simulink model "aerodynamic_model_V1_2_Wrench"  (R2025b)
settings: Solver=ode4  StartTime=0.0  StopTime=0.3  FixedStep=Ts  RelTol=1e-3
InitFcn:
  | % Run initial_main.m first to load Ad,As,Tq_prop,Tq_mass,...
values from neighbouring files (symbols this model uses):
  alpha_du0_v_tail_L = trim_aero_ic.v_tail_L.alpha_du0    [initial_main_V1_1.m]
  alpha_du0_v_tail_R = trim_aero_ic.v_tail_R.alpha_du0    [initial_main_V1_1.m]
  alpha_du0_wing_L = trim_aero_ic.wing_L.alpha_du0    [initial_main_V1_1.m]
  alpha_du0_wing_R = trim_aero_ic.wing_R.alpha_du0    [initial_main_V1_1.m]
  As = sys_sd.A    [initial_main_V1_1.m]
  BladePitch_deg = 34    [initial_main_V1_1.m]
  Bs = sys_sd.B    [initial_main_V1_1.m]
  Cs = sys_sd.C    [initial_main_V1_1.m]
  ctrl_delta_lim_deg = strips.delta_lim_deg    [initial_main_V1_1.m]
  ctrl_map_aileron_L = aero.wing_L.map_aileron(:)    [initial_main_V1_1.m]
  ctrl_map_aileron_R = aero.wing_R.map_aileron(:)    [initial_main_V1_1.m]
  ctrl_map_tail_L = aero.v_tail_L.map_tail(:)    [initial_main_V1_1.m]
  ctrl_map_tail_R = aero.v_tail_R.map_tail(:)    [initial_main_V1_1.m]
  Ds = sys_sd.D    [initial_main_V1_1.m]
  I_cg_b = R_sb * I_cg_m * R_sb.'    [aeroelastic.m]    (also in initial_main_V1_1.m = grav.I_cg_b)
  I_cg_b_inv = R_sb * I_cg_m_inv * R_sb.'    [aeroelastic.m]    (also in initial_main_V1_1.m = grav.I_cg_b_inv)
  m_node = zeros(n_id, 1)    [aeroelastic.m]    (also in generate_pullup_load_cloud.m = evalin('base', 'm_node(:)'); initial_main_V1_1.m = nodal.m_node)
  m_total_kg = evalin('base', 'm_total_kg')    [generate_pullup_load_cloud.m]    (also in initial_main_V1_1.m = grav.m_total_kg)
  n_modes = size(Phi, 2)    [aeroelastic.m]    (also in initial_main_V1_1.m = n_rigid + n_elastic)
  ones_1_tail = ones(1, size(r_cg2ac_b_v_tail_L, 2))    [initial_main_V1_1.m]
  ones_1_wing = ones(1, size(r_cg2ac_b_wing_L, 2))    [initial_main_V1_1.m]
  Phi = evalin('base', 'Phi')    [generate_pullup_load_cloud.m]    (also in initial_main_V1_1.m = strips.Phi)
  polar_alpha_deg = polar.alpha_deg(:).'    [initial_main_V1_1.m]
  polar_CD = polar.CD(:).'    [initial_main_V1_1.m]
  polar_CDp = polar.CDp(:).'    [initial_main_V1_1.m]
  polar_CL = polar.CL(:).'    [initial_main_V1_1.m]
  polar_CM = polar.CM(:).'    [initial_main_V1_1.m]
  r_cg2ac_b_v_tail_L = R_sb * aero.v_tail_L.r_ac_s    [initial_main_V1_1.m]
  r_cg2ac_b_v_tail_R = R_sb * aero.v_tail_R.r_ac_s    [initial_main_V1_1.m]
  r_cg2ac_b_wing_L = R_sb * aero.wing_L.r_ac_s    [initial_main_V1_1.m]
  r_cg2ac_b_wing_R = R_sb * aero.wing_R.r_ac_s    [initial_main_V1_1.m]
  r_cg2kink_b = eng.r_cg2kink_b    [initial_main_V1_1.m]
  r_cg2node_b = aeroelastic.node_arms(nodes, 'R_sb', R_sb).r_cg2node_b    [initial_main_V1_1.m]
  surface_nodes = aeroelastic.surface_load_nodes(nodes)    [initial_main_V1_1.m]
  T_aero2W = aeroelastic.wing_aileron_to_W(strips).T    [initial_main_V1_1.m]
  T_prop2W = load_maps.T_prop2W    [initial_main_V1_1.m]
  Tq_mass = load_maps.Tq_mass    [initial_main_V1_1.m]
  trim_Attitude_rad0 = trim_default.Attitude_rad0    [initial_main_V1_1.m]
  trim_Omega_b0 = trim_default.Omega_b0    [initial_main_V1_1.m]
  trim_Position0 = trim_default.Position0    [initial_main_V1_1.m]
  trim_Velocity_b0 = trim_default.Velocity_b0    [initial_main_V1_1.m]
  Ts = 0.001    [initial_main_V1_1.m]
  U = 55    [initial_main_V1_1.m]
  v_tail_cant_rad = deg2rad(v_tail_cant_deg)    [initial_main_V1_1.m]
  W_mass_g = grav.W_mass    [initial_main_V1_1.m]
  x0_structure = trim_default.x0_structure    [initial_main_V1_1.m]
  x0_wagner_v_tail_L = trim_aero_ic.v_tail_L.x0_wagner    [initial_main_V1_1.m]
  x0_wagner_v_tail_R = trim_aero_ic.v_tail_R.x0_wagner    [initial_main_V1_1.m]
  x0_wagner_wing_L = trim_aero_ic.wing_L.x0_wagner    [initial_main_V1_1.m]
  x0_wagner_wing_R = trim_aero_ic.wing_R.x0_wagner    [initial_main_V1_1.m]
undefined symbols (not defined in the file or in its folder): Ad_v_tail_L, Ad_v_tail_R, Ad_wing_L, Ad_wing_R, Bd_v_tail_L, Bd_v_tail_R, Bd_wing_L, Bd_wing_R, c_over_2U_v_tail_L, c_over_2U_v_tail_R, c_over_2U_wing_L, c_over_2U_wing_R, Cd_v_tail_L, Cd_v_tail_R, Cd_wing_L, Cd_wing_R, Dd_v_tail_L, Dd_v_tail_R, Dd_wing_L, Dd_wing_R, G_du_v_tail_L, G_du_v_tail_R, G_du_wing_L, G_du_wing_R, polar_aileron_alpha_deg, polar_aileron_dCD, polar_aileron_dCL, polar_aileron_dCM, polar_aileron_delta_deg, polar_ruddervator_alpha_deg, polar_ruddervator_dCD, polar_ruddervator_dCL, polar_ruddervator_dCM, polar_ruddervator_delta_deg, qS_strip_v_tail_L, qS_strip_v_tail_R, qS_strip_wing_L, qS_strip_wing_R, qSc_strip_v_tail_L, qSc_strip_v_tail_R, qSc_strip_wing_L, qSc_strip_wing_R, T_m2b_v_tail_L, T_m2b_v_tail_R, T_m2b_wing_L, T_m2b_wing_R, T_m2h_v_tail_L, T_m2h_v_tail_R, T_m2h_wing_L, T_m2h_wing_R, Tq_CM_v_tail_L, Tq_CM_v_tail_R, Tq_CM_wing_L, Tq_CM_wing_R, Tq_D_v_tail_L, Tq_D_v_tail_R, Tq_D_wing_L, Tq_D_wing_R, Tq_v_tail_L, Tq_v_tail_R ... (+2)
libraries: Prop_gryo x12, matrix_library x2
(part 1 of 6)
settings Model: Creator=someone  LastModifiedBy=someone
settings DataIOCC: ExternalInput=trim_input_dataset  LoadExternalInput=on

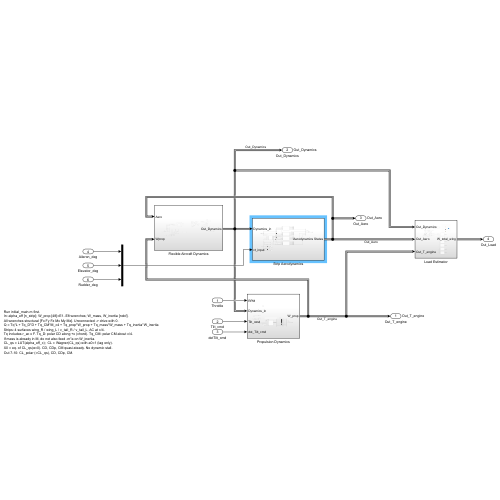
[thumbnail: Simulink's stored preview of the top-level diagram]
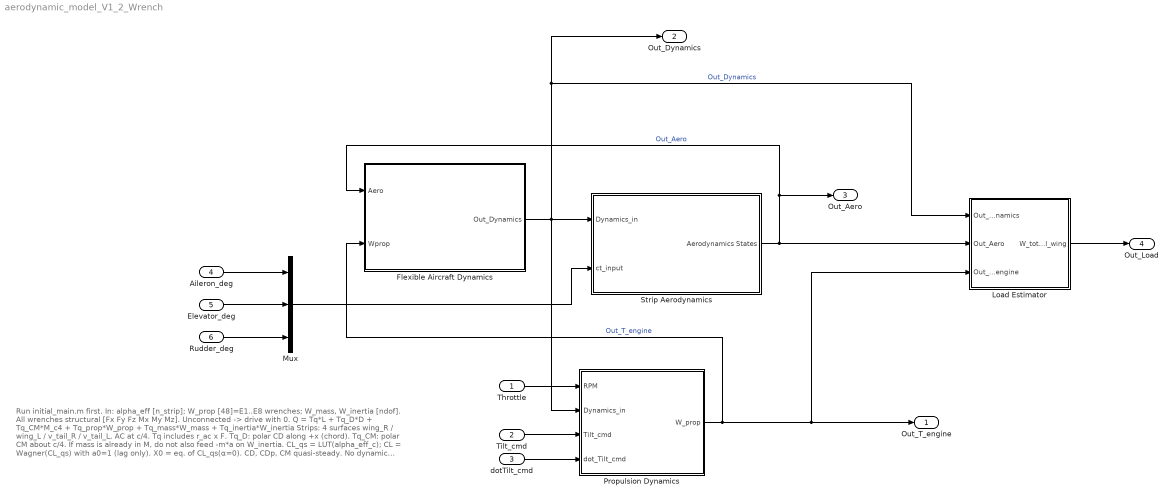
== system aerodynamic_model_V1_2_Wrench ==
  note: Run initial_main.m first.
      | In: alpha_eff [n_strip]; W_prop [48]=E1..E8 wrenches; W_mass, W_inertia [ndof].
      | All wrenches structural [Fx Fy Fz Mx My Mz]. Unconnected -> drive with 0.
      | Q = Tq*L + Tq_D*D + Tq_CM*M_c4 + Tq_prop*W_prop + Tq_mass*W_mass + Tq_inertia*W_inertia
      | Strips: 4 surfaces wing_R / wing_L / v_tail_R / v_tail_L, AC at c/4.
      | Tq includes r_ac x F. Tq_D: polar CD along +x (chord). Tq_CM: polar CM about c/4.
      | If mass is already in M, do not also feed -m*a on W_inertia.
      | CL_qs = LUT(alpha_eff_c);  CL = Wagner(CL_qs) with a0=1 (lag only).
      | X0 = eq. of CL_qs(α=0). CD, CDp, CM quasi-steady. No dynamic stall.
      | Out 7-10: CL_polar (=CL_qs), CD, CDp, CM.
  Throttle : Inport  PortDimensions=8
  Tilt_cmd : Inport  Port=2  PortDimensions=8
  dotTilt_cmd : Inport  Port=3  PortDimensions=8
  Aileron_deg : Inport  Port=4
  Elevator_deg : Inport  Port=5
  Rudder_deg : Inport  Port=6
  Flexible Aircraft Dynamics : Subsystem
  Load Estimator : Subsystem
  Mux : Mux  Inputs=3
  Propulsion Dynamics : Subsystem
  Strip Aerodynamics : Subsystem
  Out_T_engine : Outport  SignalName=Out_T_engine
  Out_Dynamics : Outport  Port=2  SignalName=Out_Dynamics
  Out_Aero : Outport  Port=3  SignalName=Out_Aero
  Out_Load : Outport  Port=4
  wires:
  Throttle/1 -> Propulsion Dynamics/1(RPM)
  Tilt_cmd/1 -> Propulsion Dynamics/3(Tilt_cmd)
  dotTilt_cmd/1 -> Propulsion Dynamics/4(dot_Tilt_cmd)
  Flexible Aircraft Dynamics/1(Out_Dynamics) -> Out_Dynamics/1, Load Estimator/1(Out_Dynamics), Strip Aerodynamics/1(Dynamics_in), Propulsion Dynamics/2(Dynamics_in)  "Out_Dynamics"
  Strip Aerodynamics/1(Aerodynamics States) -> Out_Aero/1, Flexible Aircraft Dynamics/1(Aero), Load Estimator/2(Out_Aero)  "Out_Aero"
  Propulsion Dynamics/1(W_prop) -> Load Estimator/3(Out_T_engine), Out_T_engine/1, Flexible Aircraft Dynamics/2(Wprop)  "Out_T_engine"
  Aileron_deg/1 -> Mux/1
  Rudder_deg/1 -> Mux/3
  Mux/1 -> Strip Aerodynamics/2(ct_input)
  Elevator_deg/1 -> Mux/2
  Load Estimator/1(W_total_wing) -> Out_Load/1

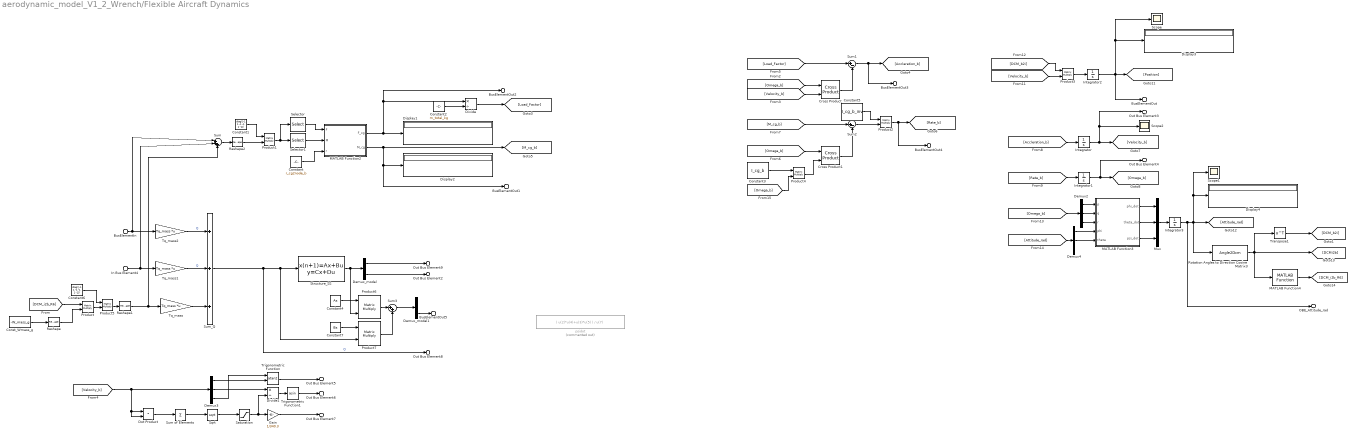
== system aerodynamic_model_V1_2_Wrench/Flexible Aircraft Dynamics ==
  BusElementIn : Inport  PortName=Aero  Element=W_aero_S
  In Bus Element4 : Inport  Port=2  PortName=Wprop  Element=W_m
  Const_Wmass_g : Constant  Value=-W_mass_g
  Constant : Constant  Value=r_cg2node_b
  Constant1 : Constant  Value=diag([-1 1 -1 -1 1 -1])
  Constant2 : Constant  Value=m_total_kg
  Constant3 : Constant  Value=I_cg_b
  Constant4 : Constant  Value=As
  Constant5 : Constant  Value=I_cg_b_inv
  Constant6 : Constant  Value=diag([-1 1 -1 -1 1 -1])
  Constant7 : Constant  Value=Bs
  Cross Product : matrix_library/Cross Product
  Cross Product1 : matrix_library/Cross Product
  Demux2 : Demux  Outputs=3
  Demux3 : Demux  Outputs=3
  Demux4 : Demux  Outputs=3
  Demux_modal : Demux  Outputs=[n_modes n_modes]
  Demux_modal1 : Demux  Outputs=[n_modes n_modes]
  Display{1..4} (4 alike) : Display
  Divide : Product  Inputs=*/
  Divide1 : Product  Inputs=*/
  Dot Product : DotProduct  OutDataTypeStr=Inherit: Inherit via internal rule
  Gain : Gain  Gain=1/340.3
  Integrator : Integrator  InitialCondition=trim_Velocity_b0
  Integrator1 : Integrator  InitialCondition=trim_Omega_b0
  Integrator2 : Integrator  InitialCondition=trim_Position0
  Integrator3 : Integrator  InitialCondition=trim_Attitude_rad0
  MATLAB Function2 : MATLAB Function  TreatAsAtomicUnit=on
  MATLAB Function3 : MATLAB Function  TreatAsAtomicUnit=on
  MATLAB Function4 : Prop_gryo/Prop1/MATLAB Function  SystemSampleTime=-1  VariantActivationTime=update diagram  EmptyChoice=off  PassThrough=off  PassThroughVariantControl=(default)  EmptyChoiceVariantControl=(default)  AllowFlexibleInterface=on  Latency=0  AutoFrameSizeCalculation=off
  Mux : Mux  Inputs=3
  Product{,1..7} (8 alike) : Product  Multiplication=Matrix(*)
  Reshape : Reshape  OutputDimensionality=Customize  OutputDimensions=[6 89]
  Reshape1 : Reshape
  Reshape2 : Reshape  OutputDimensionality=Customize  OutputDimensions=[6 89]
  Rotation Angles to Direction Cosine Matrix3 : Angle2Dcm
      settings: AttributesFormatString=Rotation Order: %<rotationOrder>
  Saturation : Saturate  UpperLimit=inf  LowerLimit=1e-6
  Scope : Scope
      settings: ActiveDisplayYMinimum=-1  ActiveDisplayYMaximum=1
  Scope1 : Scope
      settings: ActiveDisplayYMinimum=-0.70675522606206342  ActiveDisplayYMaximum=0.36695629334776858
  Scope2 : Scope
      settings: ActiveDisplayYMinimum=-1  ActiveDisplayYMaximum=1  DataLoggingVariableName=ScopeData2
  Selector : Selector  NumberOfDimensions=2  InputPortWidth=3  IndexOptions=Index vector (dialog),Index vector (dialog)  Indices=[1:3],[1:89]  OutputSizes=1,1
  Selector1 : Selector  NumberOfDimensions=2  InputPortWidth=3  IndexOptions=Index vector (dialog),Index vector (dialog)  Indices=[4:6],[1:89]  OutputSizes=1,1
  Sqrt : Sqrt
  Structure_SS : DiscreteStateSpace  A=As  B=Bs  C=Cs  D=Ds  InitialCondition=x0_structure  SampleTime=Ts
  Sum : Sum  Inputs=|+++
  Sum of Elements : Sum  Inputs=+
  Sum1 : Sum  Inputs=|+-
  Sum2 : Sum  Inputs=|+-
  Sum3 : Sum  Inputs=|++
  Sum_Q : Sum  Inputs=+++
  Tq_mass : Gain  Gain=Tq_mass  Multiplication=Matrix(K*u)
  Tq_mass1 : Gain  Gain=Tq_mass  Multiplication=Matrix(K*u)
  Tq_mass2 : Gain  Gain=Tq_mass  Multiplication=Matrix(K*u)
  Transpose1 : Math  Operator=transpose
  Trigonometric Function : Trigonometry  Operator=atan2
  Trigonometric Function1 : Trigonometry  Operator=asin
  psidot : Fcn  Commented=on  Expr=( u(2)*u(4)+u(3)*u(5) ) / u(7)
  Out Bus Element2 : Outport  PortName=Out_Dynamics  Element=elastic_m_velocity
  Out Bus Element3 : Outport  PortName=Out_Dynamics  Element=Velocity_b
  Out Bus Element4 : Outport  PortName=Out_Dynamics  Element=Omega_b
  Out Bus Element5 : Outport  PortName=Out_Dynamics  Element=Alpha
  Out Bus Element6 : Outport  PortName=Out_Dynamics  Element=Beta
  Out Bus Element7 : Outport  PortName=Out_Dynamics  Element=mach
  Out Bus Element8 : Outport  PortName=Out_Dynamics  Element=Q
  Out Bus Element9 : Outport  PortName=Out_Dynamics  Element=elastic_displacement
  OBE_Attitude_rad : Outport  PortName=Out_Dynamics  Element=Attitude_rad
  BusElementOut : Outport  PortName=Out_Dynamics  Element=Position
  BusElementOut1 : Outport  PortName=Out_Dynamics  Element=M_cg
  BusElementOut2 : Outport  PortName=Out_Dynamics  Element=F_cg
  BusElementOut3 : Outport  PortName=Out_Dynamics  Element=Acc_b
  BusElementOut4 : Outport  PortName=Out_Dynamics  Element=Rate_b
  BusElementOut5 : Outport  PortName=Out_Dynamics  Element=elastic_acc
  wires:
  Dot Product/1 -> Sum of Elements/1
  [Velocity_b] -> Demux3/1, Dot Product/2, Dot Product/1
  Demux3/3 -> Trigonometric Function/1
  Sum_Q/1 -> Product7/2, Structure_SS/1, Out Bus Element8/1  "Q"
  In Bus Element4/1 -> Tq_mass1/1, Sum/2
  Demux_modal/2 -> Out Bus Element2/1
  Demux_modal/1 -> Out Bus Element9/1
  Tq_mass/1 -> Sum_Q/3
  Sum of Elements/1 -> Sqrt/1
  Demux3/2 -> Divide1/1
  Structure_SS/1 -> Product6/2, Demux_modal/1
  Divide1/1 -> Trigonometric Function1/1
  Demux3/1 -> Trigonometric Function/2
  Const_Wmass_g/1 -> Reshape/1
  Sqrt/1 -> Saturation/1
  Saturation/1 -> Gain/1, Divide1/2
  Trigonometric Function/1 -> Out Bus Element5/1
  Trigonometric Function1/1 -> Out Bus Element6/1
  Gain/1 -> Out Bus Element7/1
  Tq_mass1/1 -> Sum_Q/2  "Q"
  BusElementIn/1 -> Sum/1, Tq_mass2/1
  Tq_mass2/1 -> Sum_Q/1  "Q"
  [DCM_i2b_R6] -> Product/1
  Reshape/1 -> Product/2
  Product5/1 -> Reshape1/1
  Reshape1/1 -> Tq_mass/1, Sum/3
  Sum/1 -> Reshape2/1
  Reshape2/1 -> Product1/2
  Selector/1 -> MATLAB Function2/1(F)
  Selector1/1 -> MATLAB Function2/2(M)
  Constant/1 -> MATLAB Function2/3(r)
  Constant1/1 -> Product1/1
  Product1/1 -> Selector1/1, Selector/1
  MATLAB Function2/1(F_cg) -> BusElementOut2/1, Divide/1, Display1/1
  MATLAB Function2/2(M_cg) -> Display2/1, BusElementOut1/1, [M_cg_b]
  [Omega_b] -> Cross Product/1
  [Velocity_b] -> Cross Product/2
  [Load_Factor] -> Sum1/1
  Cross Product/1 -> Sum1/2
  Constant2/1 -> Divide/2
  Divide/1 -> [Load_Factor]
  Sum1/1 -> BusElementOut3/1, [Accleration_b]
  [Omega_b] -> Cross Product1/1
  Constant3/1 -> Product4/1
  [M_cg_b] -> Sum2/1
  Cross Product1/1 -> Sum2/2
  [Accleration_b] -> Integrator/1
  [Rate_b] -> Integrator1/1
  Integrator/1 -> Scope2/1, Out Bus Element3/1, [Velocity_b]
  Integrator1/1 -> Out Bus Element4/1, [Omega_b]
  Sum2/1 -> Product2/2
  Constant5/1 -> Product2/1
  Product2/1 -> BusElementOut4/1, [Rate_b]
  [Velocity_b] -> Product3/2
  [DCM_b2i] -> Product3/1
  Product3/1 -> Integrator2/1
  Integrator2/1 -> BusElementOut/1, Display3/1, Scope/1, [Position]
  Integrator3/1 -> Rotation Angles to Direction Cosine Matrix3/1, Scope1/1, Display4/1, [Attitude_rad], OBE_Attitude_rad/1
  [Omega_b] -> Demux2/1
  Demux2/1 -> MATLAB Function3/1(p)
  Demux2/2 -> MATLAB Function3/2(q)
  Demux2/3 -> MATLAB Function3/3(r)
  [Attitude_rad] -> Demux4/1
  Demux4/1 -> MATLAB Function3/4(phi)
  Demux4/2 -> MATLAB Function3/5(theta)
  Mux/1 -> Integrator3/1
  MATLAB Function3/1(phi_dot) -> Mux/1
  MATLAB Function3/2(theta_dot) -> Mux/2
  MATLAB Function3/3(psi_dot) -> Mux/3
  [Omega_b] -> Product4/2
  Product4/1 -> Cross Product1/2
  Rotation Angles to Direction Cosine Matrix3/1 -> Transpose1/1, MATLAB Function4/1, [DCMi2b]
  MATLAB Function4/1 -> [DCM_i2b_R6]
  Transpose1/1 -> [DCM_b2i]
  Constant6/1 -> Product5/1
  Product/1 -> Product5/2
  Product6/1 -> Sum3/1
  Product7/1 -> Sum3/2
  Constant4/1 -> Product6/1
  Constant7/1 -> Product7/1
  Sum3/1 -> Demux_modal1/1
  Demux_modal1/2 -> BusElementOut5/1

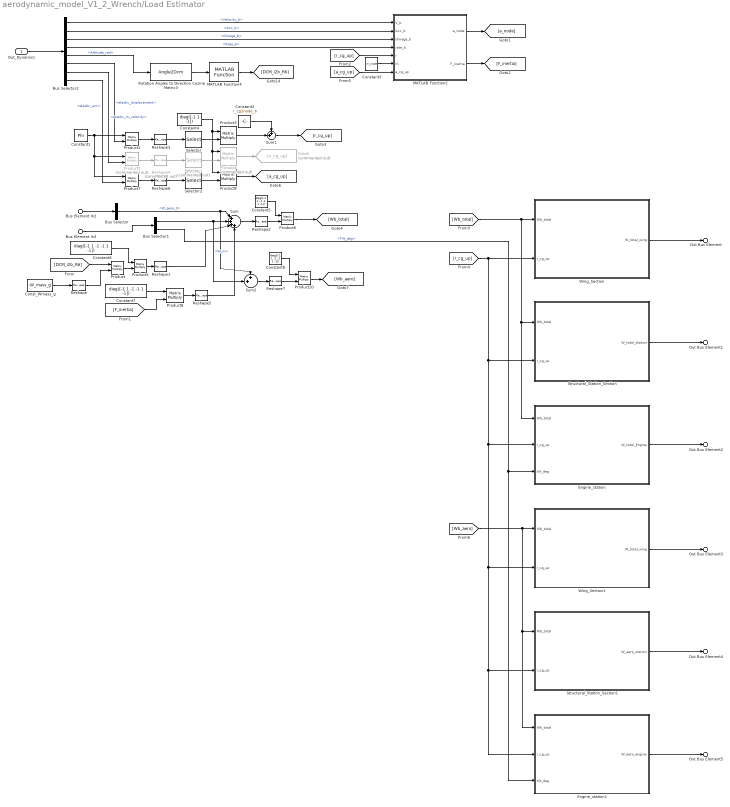
== system aerodynamic_model_V1_2_Wrench/Load Estimator ==
  Out_Dynamics : Inport
  Bus Element In2 : Inport  Port=2  PortName=Out_Aero
  Bus Element In3 : Inport  Port=3  PortName=Out_T_engine
  Bus Selector : BusSelector  OutputSignals=W_aero_S
  Bus Selector1 : BusSelector  OutputSignals=W_m,Tilt_deg
  Bus Selector2 : BusSelector  OutputSignals=Velocity_b,Acc_b,Omega_b,Rate_b,Attitude_rad,elastic_displacement,elastic_m_velocity,elastic_acc
  Const_Wmass_g : Constant  Value=-W_mass_g
  Constant1 : Constant  Value=Phi
  Constant2 : Constant  Value=r_cg2node_b
  Constant3 : Constant  Value=m_node
  Constant4 : Constant  Value=diag([-1 1 -1])
  Constant{5..8} (4 alike) : Constant  Value=diag([-1 1 -1 -1 1 -1])
  Engine_station : Subsystem
  Engine_station1 : Subsystem
  Goto5 : Goto  Commented=on  GotoTag=v_cg_up
  MATLAB Function2 : MATLAB Function  TreatAsAtomicUnit=on
  MATLAB Function4 : Prop_gryo/Prop1/MATLAB Function  SystemSampleTime=-1  VariantActivationTime=update diagram  EmptyChoice=off  PassThrough=off  PassThroughVariantControl=(default)  EmptyChoiceVariantControl=(default)  AllowFlexibleInterface=on  Latency=0  AutoFrameSizeCalculation=off
  Product{,1,3,5..10} (9 alike) : Product  Multiplication=Matrix(*)
  Product2 : Product  Commented=on  Multiplication=Matrix(*)
  Product4 : Product  Commented=on  Multiplication=Matrix(*)
  Reshape{,2..3,6..7} (5 alike) : Reshape  OutputDimensionality=Customize  OutputDimensions=[6 89]
  Reshape1 : Reshape
  Reshape4 : Reshape  Commented=on  OutputDimensionality=Customize  OutputDimensions=[6 89]
  Reshape5 : Reshape
  Rotation Angles to Direction Cosine Matrix3 : Angle2Dcm
      settings: AttributesFormatString=Rotation Order: %<rotationOrder>
  Selector : Selector  NumberOfDimensions=2  InputPortWidth=89  IndexOptions=Index vector (dialog),Index vector (dialog)  Indices=[1:3],[1:89]  OutputSizes=1,1
  Selector1 : Selector  Commented=on  NumberOfDimensions=2  InputPortWidth=89  IndexOptions=Index vector (dialog),Index vector (dialog)  Indices=[1:3],[1:89]  OutputSizes=1,1
  Selector2 : Selector  NumberOfDimensions=2  InputPortWidth=89  IndexOptions=Index vector (dialog),Index vector (dialog)  Indices=[1:3],[1:89]  OutputSizes=1,1
  Structural_Station_Section : Subsystem
  Structural_Station_Section1 : Subsystem
  Sum : Sum  Inputs=|++++
  Sum1 : Sum  Inputs=++|
  Sum2 : Sum  Inputs=++|
  Wing_Section : Subsystem
  Wing_Section1 : Subsystem
  Out Bus Element : Outport  PortName=W_total_wing  Element=W_total_wing
  Out Bus Element1 : Outport  PortName=W_total_wing  Element=W_total_station
  Out Bus Element2 : Outport  PortName=W_total_wing  Element=W_total_engine
  Out Bus Element3 : Outport  PortName=W_total_wing  Element=W_aero_wing
  Out Bus Element4 : Outport  PortName=W_total_wing  Element=W_aero_station
  Out Bus Element5 : Outport  PortName=W_total_wing  Element=W_aero_engine
  wires:
  Sum/1 -> Reshape2/1
  Bus Selector1/1 -> Sum2/2, Sum/2  "<W_m>"
  Bus Selector/1 -> Sum/1, Sum2/1  "<W_aero_S>"
  Reshape1/1 -> Sum/3
  Bus Element In2/1 -> Bus Selector/1
  Bus Element In3/1 -> Bus Selector1/1
  Reshape/1 -> Product/2
  Const_Wmass_g/1 -> Reshape/1
  [DCM_i2b_R6] -> Product/1
  Constant6/1 -> Product5/1
  Product5/1 -> Reshape1/1
  Product/1 -> Product5/2
  Out_Dynamics/1 -> Bus Selector2/1
  Bus Selector2/1 -> MATLAB Function2/1(V_b)  "<Velocity_b>"
  Bus Selector2/3 -> MATLAB Function2/3(Omega_b)  "<Omega_b>"
  Bus Selector2/2 -> MATLAB Function2/2(Acc_b)  "<Acc_b>"
  [r_cg_up] -> MATLAB Function2/5(r)
  Bus Selector2/4 -> MATLAB Function2/4(rate_b)  "<Rate_b>"
  Constant3/1 -> MATLAB Function2/6(m)
  Rotation Angles to Direction Cosine Matrix3/1 -> MATLAB Function4/1
  Bus Selector2/5 -> Rotation Angles to Direction Cosine Matrix3/1  "<Attitude_rad>"
  MATLAB Function4/1 -> [DCM_i2b_R6]
  MATLAB Function2/1(a_node) -> [a_node]
  MATLAB Function2/2(F_inertia) -> [F_inertia]
  Reshape5/1 -> Sum/4
  Bus Selector2/6 -> Product1/2  "<elastic_displacement>"
  Constant1/1 -> Product1/1, Product2/1, Product7/1
  Bus Selector2/7 -> Product2/2  "<elastic_m_velocity>"
  Product1/1 -> Reshape3/1
  Product2/1 -> Reshape4/1
  Reshape3/1 -> Selector/1
  Reshape4/1 -> Selector1/1
  Selector/1 -> Product3/2
  Constant4/1 -> Product8/1, Product4/1, Product3/1
  Selector1/1 -> Product4/2
  Constant2/1 -> Sum1/1
  Sum1/1 -> [r_cg_up]
  Product3/1 -> Sum1/2
  Product9/1 -> Reshape5/1
  Reshape2/1 -> Product6/2
  Product4/1 -> Goto5/1
  [a_cg_up] -> MATLAB Function2/7(a_cg_up)
  [Wb_total] -> Engine_station/1(Wb_total), Structural_Station_Section/1(Wb_total), Wing_Section/1(Wb_total)
  [r_cg_up] -> Structural_Station_Section/2(r_cg_up), Wing_Section1/2(r_cg_up), Engine_station1/2(r_cg_up), Structural_Station_Section1/2(r_cg_up), Engine_station/2(r_cg_up), Wing_Section/2(r_cg_up)
  Wing_Section/1(W_total_wing) -> Out Bus Element/1
  Structural_Station_Section/1(W_total_station) -> Out Bus Element1/1
  Engine_station/1(W_total_Engine) -> Out Bus Element2/1
  Bus Selector1/2 -> Engine_station/3(tilt_deg), Engine_station1/3(tilt_deg)  "<Tilt_deg>"
  Constant5/1 -> Product6/1
  Product6/1 -> [Wb_total]
  Product8/1 -> [a_cg_up]
  Selector2/1 -> Product8/2
  Reshape6/1 -> Selector2/1
  Product7/1 -> Reshape6/1
  Bus Selector2/8 -> Product7/2  "<elastic_acc>"
  [F_inertia] -> Product9/2
  Constant7/1 -> Product9/1
  Product10/1 -> [Wb_aero]
  Constant8/1 -> Product10/1
  Reshape7/1 -> Product10/2
  Sum2/1 -> Reshape7/1
  [Wb_aero] -> Wing_Section1/1(Wb_total), Engine_station1/1(Wb_total), Structural_Station_Section1/1(Wb_total)
  Wing_Section1/1(W_total_wing) -> Out Bus Element3/1
  Structural_Station_Section1/1(W_aero_station) -> Out Bus Element4/1
  Engine_station1/1(W_aero_engine) -> Out Bus Element5/1

== system aerodynamic_model_V1_2_Wrench/Propulsion Dynamics ==
  note: 根据体轴速度、加速度、引擎和铰链位置以及铰链轴和倾转角速率计算各个引擎体轴下绝对速度
  RPM : Inport  PortDimensions=8
  Dynamics_in : Inport  Port=2
  Tilt_cmd : Inport  Port=3  PortDimensions=8
  dot_Tilt_cmd : Inport  Port=4  PortDimensions=8
  BladePitch_deg : Constant  Value=BladePitch_deg
  Bus Selector : BusSelector  OutputSignals=signal1.Wb,signal2.Wb,signal3.Wb,signal4.Wb,signal5.Wb,signal6.Wb,signal7.Wb,signal8.Wb
  BusSel_Dynamic : BusSelector  OutputSignals=mach,Velocity_b,Omega_b
  Constant : Constant  Value=diag([-1 1 1 -1 1 1])
  Constant1 : Constant  Value=T_prop2W
  Constant4 : Constant  Commented=on  Value=(pi/2)*ones(8,1)
  Delay_Dynamic : UnitDelay  Commented=through  SampleTime=Ts  HasFrameUpgradeWarning=on
  Gain : Gain  Gain=1/60
  Mux1 : Mux  Inputs=8
  Product{,1..8} (9 alike) : Product  Multiplication=Matrix(*)
  Subsystem8 : Subsystem
  Out Bus Element1 : Outport  PortName=W_prop  Element=W_m
  BusElementOut : Outport  PortName=W_prop  Element=Tilt_deg
  wires:
  Dynamics_in/1 -> Delay_Dynamic/1
  Delay_Dynamic/1 -> BusSel_Dynamic/1
  BusSel_Dynamic/2 -> Subsystem8/3(Vb)  "<Velocity_b>"
  BusSel_Dynamic/3 -> Subsystem8/4(Omegab)  "<Omega_b>"
  RPM/1 -> [RPM], Gain/1
  Gain/1 -> [RPS]
  BladePitch_deg/1 -> [BladePitchAngle_DEG]
  Tilt_cmd/1 -> BusElementOut/1, Subsystem8/1(In1)
  dot_Tilt_cmd/1 -> Subsystem8/2(In2)
  [BladePitchAngle_DEG] -> Subsystem8/5(BladePitchAngle_DEG)
  [RPS] -> Subsystem8/6(RPS)
  Subsystem8/1(Prop) -> Bus Selector/1
  Constant/1 -> Product7/1, Product6/1, Product5/1, Product4/1, Product3/1, Product2/1, Product1/1, Product/1
  Bus Selector/8 -> Product7/2  "<Wb>"
  Bus Selector/7 -> Product6/2  "<Wb>"
  Bus Selector/6 -> Product5/2  "<Wb>"
  Bus Selector/5 -> Product4/2  "<Wb>"
  Bus Selector/4 -> Product3/2  "<Wb>"
  Bus Selector/3 -> Product2/2  "<Wb>"
  Bus Selector/2 -> Product1/2  "<Wb>"
  Product/1 -> Mux1/1
  Product1/1 -> Mux1/2
  Product2/1 -> Mux1/3
  Product3/1 -> Mux1/4
  Product4/1 -> Mux1/5
  Product5/1 -> Mux1/6
  Product6/1 -> Mux1/7
  Product7/1 -> Mux1/8
  Mux1/1 -> Product8/2
  Constant1/1 -> Product8/1
  Product8/1 -> Out Bus Element1/1
  Bus Selector/1 -> Product/2  "<Wb>"

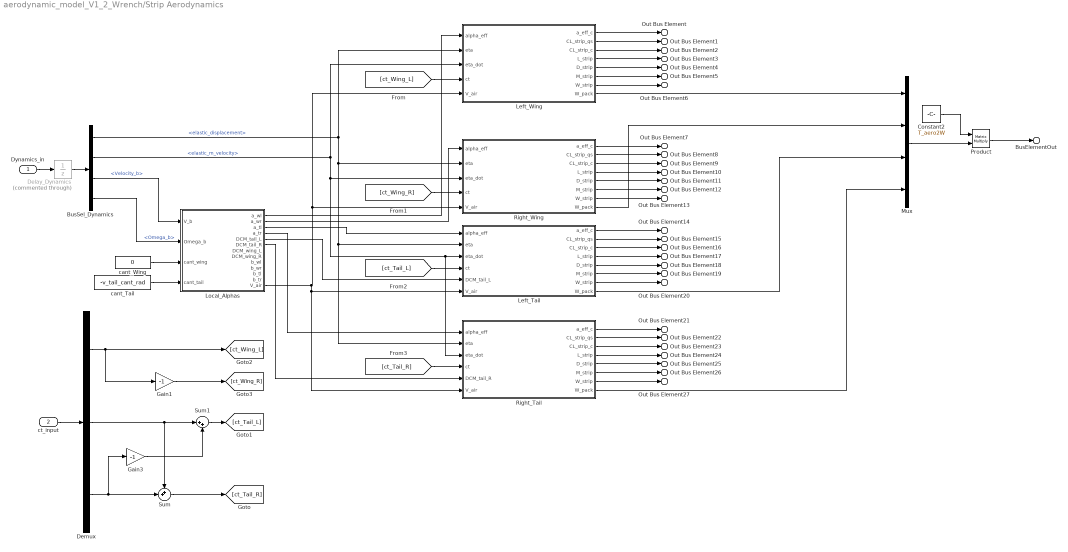
== system aerodynamic_model_V1_2_Wrench/Strip Aerodynamics ==
  Dynamics_in : Inport
  ct_input : Inport  Port=2
  BusSel_Dynamics : BusSelector  OutputSignals=elastic_displacement,elastic_m_velocity,Velocity_b,Omega_b
  Constant2 : Constant  Value=T_aero2W
  Delay_Dynamics : UnitDelay  Commented=through  SampleTime=Ts  HasFrameUpgradeWarning=on
  Demux : Demux  Outputs=3
  Gain1 : Gain  Gain=-1
  Gain3 : Gain  Gain=-1
  Left_Tail : Subsystem
  Left_Wing : Subsystem
  Local_Alphas : Subsystem
  Mux : Mux
  Product : Product  Multiplication=Matrix(*)
  Right_Tail : Subsystem
  Right_Wing : Subsystem
  Sum : Sum  Inputs=++|
  Sum1 : Sum  Inputs=|++
  cant_Tail : Constant  Value=-v_tail_cant_rad
  cant_Wing : Constant  Value=0
  Out Bus Element : Outport  PortName=Aerodynamics States  Element=a_eff_c_LW
  Out Bus Element1 : Outport  PortName=Aerodynamics States  Element=CL_strip_qs_LW
  Out Bus Element2 : Outport  PortName=Aerodynamics States  Element=CL_strip_c_LW
  Out Bus Element3 : Outport  PortName=Aerodynamics States  Element=L_strip_LW
  Out Bus Element4 : Outport  PortName=Aerodynamics States  Element=D_strip_LW
  Out Bus Element5 : Outport  PortName=Aerodynamics States  Element=M_strip_LW
  Out Bus Element6 : Outport  PortName=Aerodynamics States  Element=W_strip_LW
  Out Bus Element7 : Outport  PortName=Aerodynamics States  Element=a_eff_c_RW
  Out Bus Element8 : Outport  PortName=Aerodynamics States  Element=CL_strip_qs_RW
  Out Bus Element9 : Outport  PortName=Aerodynamics States  Element=CL_strip_c_RW
  Out Bus Element10 : Outport  PortName=Aerodynamics States  Element=L_strip_RW
  Out Bus Element11 : Outport  PortName=Aerodynamics States  Element=D_strip_RW
  Out Bus Element12 : Outport  PortName=Aerodynamics States  Element=M_strip_RW
  Out Bus Element13 : Outport  PortName=Aerodynamics States  Element=W_strip_RW
  Out Bus Element14 : Outport  PortName=Aerodynamics States  Element=a_eff_c_LT
  Out Bus Element15 : Outport  PortName=Aerodynamics States  Element=CL_strip_qs_LT
  Out Bus Element16 : Outport  PortName=Aerodynamics States  Element=CL_strip_c_LT
  Out Bus Element17 : Outport  PortName=Aerodynamics States  Element=L_strip_LT
  Out Bus Element18 : Outport  PortName=Aerodynamics States  Element=D_strip_LT
  Out Bus Element19 : Outport  PortName=Aerodynamics States  Element=M_strip_LT
  Out Bus Element20 : Outport  PortName=Aerodynamics States  Element=W_strip_LT
  Out Bus Element21 : Outport  PortName=Aerodynamics States  Element=a_eff_c_RT
  Out Bus Element22 : Outport  PortName=Aerodynamics States  Element=CL_strip_qs_RT
  Out Bus Element23 : Outport  PortName=Aerodynamics States  Element=CL_strip_c_RT
  Out Bus Element24 : Outport  PortName=Aerodynamics States  Element=L_strip_RT
  Out Bus Element25 : Outport  PortName=Aerodynamics States  Element=D_strip_RT
  Out Bus Element26 : Outport  PortName=Aerodynamics States  Element=M_strip_RT
  Out Bus Element27 : Outport  PortName=Aerodynamics States  Element=W_strip_RT
  BusElementOut : Outport  PortName=Aerodynamics States  Element=W_aero_S
  wires:
  Left_Wing/6(M_strip) -> Out Bus Element5/1
  Left_Wing/5(D_strip) -> Out Bus Element4/1
  Left_Wing/4(L_strip) -> Out Bus Element3/1
  Left_Wing/3(CL_strip_c) -> Out Bus Element2/1
  Left_Wing/2(CL_strip_qs) -> Out Bus Element1/1
  Left_Wing/1(a_eff_c) -> Out Bus Element/1
  Left_Wing/7(W_strip) -> Out Bus Element6/1
  Right_Wing/7(W_strip) -> Out Bus Element13/1
  Right_Wing/6(M_strip) -> Out Bus Element12/1
  Right_Wing/5(D_strip) -> Out Bus Element11/1
  Right_Wing/4(L_strip) -> Out Bus Element10/1
  Right_Wing/3(CL_strip_c) -> Out Bus Element9/1
  Right_Wing/2(CL_strip_qs) -> Out Bus Element8/1
  Right_Wing/1(a_eff_c) -> Out Bus Element7/1
  Left_Tail/7(W_strip) -> Out Bus Element20/1
  Left_Tail/6(M_strip) -> Out Bus Element19/1
  Left_Tail/5(D_strip) -> Out Bus Element18/1
  Left_Tail/4(L_strip) -> Out Bus Element17/1
  Left_Tail/3(CL_strip_c) -> Out Bus Element16/1
  Left_Tail/2(CL_strip_qs) -> Out Bus Element15/1
  Left_Tail/1(a_eff_c) -> Out Bus Element14/1
  Right_Tail/7(W_strip) -> Out Bus Element27/1
  Right_Tail/6(M_strip) -> Out Bus Element26/1
  Right_Tail/5(D_strip) -> Out Bus Element25/1
  Right_Tail/4(L_strip) -> Out Bus Element24/1
  Right_Tail/3(CL_strip_c) -> Out Bus Element23/1
  Right_Tail/2(CL_strip_qs) -> Out Bus Element22/1
  Right_Tail/1(a_eff_c) -> Out Bus Element21/1
  Dynamics_in/1 -> Delay_Dynamics/1
  Delay_Dynamics/1 -> BusSel_Dynamics/1
  BusSel_Dynamics/1 -> Left_Wing/2(eta), Right_Tail/2(eta), Left_Tail/2(eta), Right_Wing/2(eta)  "<elastic_displacement>"
  BusSel_Dynamics/2 -> Right_Tail/3(eta_dot), Left_Tail/3(eta_dot), Right_Wing/3(eta_dot), Left_Wing/3(eta_dot)  "<elastic_m_velocity>"
  BusSel_Dynamics/3 -> Local_Alphas/1(V_b)  "<Velocity_b>"
  cant_Wing/1 -> Local_Alphas/3(cant_wing)
  Local_Alphas/1(a_wl) -> Left_Wing/1(alpha_eff)
  Local_Alphas/2(a_wr) -> Right_Wing/1(alpha_eff)
  Local_Alphas/3(a_tl) -> Left_Tail/1(alpha_eff)
  Local_Alphas/4(a_tr) -> Right_Tail/1(alpha_eff)
  ct_input/1 -> Demux/1
  Demux/2 -> Sum/1, Sum1/1
  Sum/1 -> [ct_Tail_R]
  Sum1/1 -> [ct_Tail_L]
  [ct_Wing_L] -> Left_Wing/4(ct)
  [ct_Wing_R] -> Right_Wing/4(ct)
  [ct_Tail_L] -> Left_Tail/4(ct)
  [ct_Tail_R] -> Right_Tail/4(ct)
  Local_Alphas/5(DCM_tail_L) -> Left_Tail/5(DCM_tail_L)
  Local_Alphas/6(DCM_tail_R) -> Right_Tail/5(DCM_tail_R)
  Demux/3 -> Gain3/1, Sum/2
  Gain3/1 -> Sum1/2
  cant_Tail/1 -> Local_Alphas/4(cant_tail)
  Left_Wing/8(W_pack) -> Mux/1
  Mux/1 -> Product/2
  Right_Wing/8(W_pack) -> Mux/2
  Left_Tail/8(W_pack) -> Mux/3
  Right_Tail/8(W_pack) -> Mux/4
  Product/1 -> BusElementOut/1
  Constant2/1 -> Product/1
  BusSel_Dynamics/4 -> Local_Alphas/2(Omega_b)  "<Omega_b>"
  Demux/1 -> Gain1/1, [ct_Wing_L]
  Gain1/1 -> [ct_Wing_R]
  Local_Alphas/13(V_air) -> Left_Tail/6(V_air), Right_Tail/6(V_air), Right_Wing/5(V_air), Left_Wing/5(V_air)

== system aerodynamic_model_V1_2_Wrench/Load Estimator/Engine_station ==
  Wb_total : Inport
  r_cg_up : Inport  Port=2
  tilt_deg : Inport  Port=3
  Bus Creator : BusCreator  Inputs=8
  Demux : Demux  Outputs=8
  Subsystem : Subsystem
  Subsystem1 : Subsystem
  Subsystem2 : Subsystem
  Subsystem3 : Subsystem
  Subsystem4 : Subsystem
  Subsystem5 : Subsystem
  Subsystem6 : Subsystem
  Subsystem7 : Subsystem
  W_total_Engine : Outport
  wires:
  tilt_deg/1 -> Demux/1
  Wb_total/1 -> Subsystem4/1(In1), Subsystem7/1(In1), Subsystem6/1(Wb_total), Subsystem5/1(Wb_total), Subsystem3/1(In1), Subsystem2/1(Wb_total), Subsystem1/1(Wb_total), Subsystem/1(In1)
  r_cg_up/1 -> Subsystem4/2(r_cg_up), Subsystem7/2(r_cg_up), Subsystem6/2(r_cg_up), Subsystem5/2(r_cg_up), Subsystem3/2(r_cg_up), Subsystem2/2(r_cg_up), Subsystem1/2(r_cg_up), Subsystem/2(In2)
  Subsystem/1(Out1) -> Bus Creator/1
  Demux/2 -> Subsystem1/3(tilt_deg)
  Demux/3 -> Subsystem2/3(In3)
  Demux/7 -> Subsystem6/3(tilt_deg)
  Demux/6 -> Subsystem5/3(tilt_deg)
  Bus Creator/1 -> W_total_Engine/1
  Subsystem1/1(Out1) -> Bus Creator/2
  Subsystem2/1(Out1) -> Bus Creator/3
  Subsystem3/1(Out1) -> Bus Creator/4
  Subsystem4/1(Out1) -> Bus Creator/5
  Subsystem5/1(Out1) -> Bus Creator/6
  Subsystem6/1(Out1) -> Bus Creator/7
  Subsystem7/1(Out1) -> Bus Creator/8

== system aerodynamic_model_V1_2_Wrench/Load Estimator/Engine_station1 ==
  Wb_total : Inport
  r_cg_up : Inport  Port=2
  tilt_deg : Inport  Port=3
  Bus Creator : BusCreator  Inputs=8
  Demux : Demux  Outputs=8
  Subsystem : Subsystem
  Subsystem1 : Subsystem
  Subsystem2 : Subsystem
  Subsystem3 : Subsystem
  Subsystem4 : Subsystem
  Subsystem5 : Subsystem
  Subsystem6 : Subsystem
  Subsystem7 : Subsystem
  W_aero_engine : Outport
  wires:
  Subsystem7/1(Out1) -> Bus Creator/8
  Subsystem6/1(Out1) -> Bus Creator/7
  Subsystem5/1(Out1) -> Bus Creator/6
  Subsystem4/1(Out1) -> Bus Creator/5
  Subsystem3/1(Out1) -> Bus Creator/4
  Subsystem2/1(Out1) -> Bus Creator/3
  Subsystem1/1(Out1) -> Bus Creator/2
  Bus Creator/1 -> W_aero_engine/1
  Demux/6 -> Subsystem5/3(tilt_deg)
  Demux/7 -> Subsystem6/3(tilt_deg)
  Demux/3 -> Subsystem2/3(In3)
  Demux/2 -> Subsystem1/3(tilt_deg)
  Subsystem/1(Out1) -> Bus Creator/1
  r_cg_up/1 -> Subsystem/2(In2), Subsystem1/2(r_cg_up), Subsystem2/2(r_cg_up), Subsystem3/2(r_cg_up), Subsystem5/2(r_cg_up), Subsystem6/2(r_cg_up), Subsystem7/2(r_cg_up), Subsystem4/2(r_cg_up)
  Wb_total/1 -> Subsystem/1(In1), Subsystem1/1(Wb_total), Subsystem2/1(Wb_total), Subsystem3/1(In1), Subsystem5/1(Wb_total), Subsystem6/1(Wb_total), Subsystem7/1(In1), Subsystem4/1(In1)
  tilt_deg/1 -> Demux/1

== system aerodynamic_model_V1_2_Wrench/Load Estimator/Structural_Station_Section ==
  Wb_total : Inport
  r_cg_up : Inport  Port=2
  Bus Creator : BusCreator  Inputs=6
  Bus Creator1 : BusCreator  Inputs=6
  Bus Creator2 : BusCreator  Inputs=6
  Bus Creator3 : BusCreator  Inputs=3
  Constant : Constant  Value=r_cg2node_b(:,7)
  Constant1 : Constant  Value=r_cg2node_b(:,13)
  Constant2 : Constant  Value=[0 0 0]/180*pi
  Constant3 : Constant  Value=r_cg2node_b(:,14)
  Constant4 : Constant  Value=[0 0 0]/180*pi
  Constant5 : Constant  Value=[0 0 0]/180*pi
  Demux{1..6} (6 alike) : Demux  Outputs=3
  MATLAB Function1 : MATLAB Function  TreatAsAtomicUnit=on
  MATLAB Function2 : MATLAB Function  TreatAsAtomicUnit=on
  MATLAB Function3 : MATLAB Function  TreatAsAtomicUnit=on
  Product{1..4,6..7} (6 alike) : Product  Multiplication=Matrix(*)
  Rotation Angles to Direction Cosine Matrix : Angle2Dcm  rotationOrder=XYZ
      settings: AttributesFormatString=Rotation Order: %<rotationOrder>
  Rotation Angles to Direction Cosine Matrix1 : Angle2Dcm  rotationOrder=XYZ
      settings: AttributesFormatString=Rotation Order: %<rotationOrder>
  Rotation Angles to Direction Cosine Matrix2 : Angle2Dcm  rotationOrder=XYZ
      settings: AttributesFormatString=Rotation Order: %<rotationOrder>
  Selector1 : Selector  NumberOfDimensions=2  InputPortWidth=3  IndexOptions=Select all,Index vector (dialog)  Indices=[1:6],[surface_nodes.v_tail_joint.node_id]  OutputSizes=1,1
  Selector10 : Selector  NumberOfDimensions=2  InputPortWidth=3  IndexOptions=Index vector (dialog),Select all  Indices=[4:6],[surface_nodes.wing_R.node_id]  OutputSizes=1,1
  Selector11 : Selector  NumberOfDimensions=2  InputPortWidth=3  IndexOptions=Index vector (dialog),Select all  Indices=[4:6],[surface_nodes.wing_R.node_id]  OutputSizes=1,1
  Selector12 : Selector  NumberOfDimensions=2  InputPortWidth=3  IndexOptions=Index vector (dialog),Select all  Indices=[1:3],[surface_nodes.wing_R.node_id]  OutputSizes=1,1
  Selector13 : Selector  NumberOfDimensions=2  InputPortWidth=3  IndexOptions=Index vector (dialog),Select all  Indices=[4:6],[surface_nodes.wing_R.node_id]  OutputSizes=1,1
  Selector14 : Selector  NumberOfDimensions=2  InputPortWidth=3  IndexOptions=Index vector (dialog),Select all  Indices=[1:3],[surface_nodes.wing_R.node_id]  OutputSizes=1,1
  Selector2 : Selector  NumberOfDimensions=2  InputPortWidth=3  IndexOptions=Select all,Index vector (dialog)  Indices=[1:6],[surface_nodes.wing_joint.node_id]  OutputSizes=1,1
  Selector3 : Selector  NumberOfDimensions=2  InputPortWidth=3  IndexOptions=Select all,Index vector (dialog)  Indices=[1:6],[surface_nodes.wing_joint.node_id]  OutputSizes=1,1
  Selector4 : Selector  NumberOfDimensions=2  InputPortWidth=3  IndexOptions=Select all,Index vector (dialog)  Indices=[1:6],[surface_nodes.v_tail_joint.node_id]  OutputSizes=1,1
  Selector5 : Selector  NumberOfDimensions=2  InputPortWidth=3  IndexOptions=Select all,Index vector (dialog)  Indices=[1:6],surface_nodes.tail_bay.node_id  OutputSizes=1,1
  Selector6 : Selector  NumberOfDimensions=2  InputPortWidth=3  IndexOptions=Select all,Index vector (dialog)  Indices=[1:6],surface_nodes.tail_bay.node_id  OutputSizes=1,1
  Selector9 : Selector  NumberOfDimensions=2  InputPortWidth=3  IndexOptions=Index vector (dialog),Select all  Indices=[1:3],[surface_nodes.wing_R.node_id]  OutputSizes=1,1
  W_total_station : Outport
  wires:
  r_cg_up/1 -> Selector6/1, Selector4/1, Selector3/1
  Wb_total/1 -> Selector2/1, Selector1/1, Selector5/1
  MATLAB Function3/2(M_b) -> Product4/2
  Rotation Angles to Direction Cosine Matrix2/1 -> Product3/1, Product4/1
  Constant3/1 -> MATLAB Function3/4(p)
  Selector6/1 -> MATLAB Function3/3(r)
  MATLAB Function3/1(F_b) -> Product3/2
  Constant4/1 -> Rotation Angles to Direction Cosine Matrix2/1
  Constant2/1 -> Rotation Angles to Direction Cosine Matrix1/1
  MATLAB Function2/1(F_b) -> Product1/2
  Selector4/1 -> MATLAB Function2/3(r)
  Constant1/1 -> MATLAB Function2/4(p)
  Rotation Angles to Direction Cosine Matrix1/1 -> Product2/1, Product1/1
  MATLAB Function2/2(M_b) -> Product2/2
  MATLAB Function1/2(M_b) -> Product7/2
  Rotation Angles to Direction Cosine Matrix/1 -> Product6/1, Product7/1
  Constant/1 -> MATLAB Function1/4(p)
  Selector3/1 -> MATLAB Function1/3(r)
  MATLAB Function1/1(F_b) -> Product6/2
  Constant5/1 -> Rotation Angles to Direction Cosine Matrix/1
  Selector10/1 -> MATLAB Function1/2(M)
  Selector9/1 -> MATLAB Function1/1(F)
  Selector2/1 -> Selector10/1, Selector9/1
  Selector12/1 -> MATLAB Function2/1(F)
  Selector11/1 -> MATLAB Function2/2(M)
  Selector1/1 -> Selector11/1, Selector12/1
  Selector5/1 -> Selector13/1, Selector14/1
  Selector13/1 -> MATLAB Function3/2(M)
  Selector14/1 -> MATLAB Function3/1(F)
  Demux4/1 -> Bus Creator/1  "Axial_Force"
  Demux5/2 -> Bus Creator/5  "Bending_momentx"
  Demux4/2 -> Bus Creator/2  "shear_forcey"
  Demux5/3 -> Bus Creator/6  "Bending_momenty"
  Product7/1 -> Demux5/1
  Product6/1 -> Demux4/1
  Demux4/3 -> Bus Creator/3  "shear_forcez"
  Demux5/1 -> Bus Creator/4  "Torision_moment"
  Demux2/3 -> Bus Creator1/6  "Bending_momenty"
  Product1/1 -> Demux1/1
  Demux1/2 -> Bus Creator1/2  "shear_forcey"
  Demux1/3 -> Bus Creator1/3  "shear_forcez"
  Demux1/1 -> Bus Creator1/1  "Axial_Force"
  Demux2/2 -> Bus Creator1/5  "Bending_momentx"
  Demux2/1 -> Bus Creator1/4  "Torision_moment"
  Product2/1 -> Demux2/1
  Product4/1 -> Demux6/1
  Demux6/1 -> Bus Creator2/4  "Torision_moment"
  Demux6/2 -> Bus Creator2/5  "Bending_momentx"
  Demux3/1 -> Bus Creator2/1  "Axial_Force"
  Demux3/3 -> Bus Creator2/3  "shear_forcez"
  Demux3/2 -> Bus Creator2/2  "shear_forcey"
  Product3/1 -> Demux3/1
  Demux6/3 -> Bus Creator2/6  "Bending_momenty"
  Bus Creator/1 -> Bus Creator3/1
  Bus Creator1/1 -> Bus Creator3/2
  Bus Creator2/1 -> Bus Creator3/3
  Bus Creator3/1 -> W_total_station/1

== system aerodynamic_model_V1_2_Wrench/Load Estimator/Structural_Station_Section1 ==
  Wb_total : Inport
  r_cg_up : Inport  Port=2
  Bus Creator : BusCreator  Inputs=6
  Bus Creator1 : BusCreator  Inputs=6
  Bus Creator2 : BusCreator  Inputs=6
  Bus Creator3 : BusCreator  Inputs=3
  Constant : Constant  Value=r_cg2node_b(:,7)
  Constant1 : Constant  Value=r_cg2node_b(:,13)
  Constant2 : Constant  Value=[0 0 0]/180*pi
  Constant3 : Constant  Value=r_cg2node_b(:,14)
  Constant4 : Constant  Value=[0 0 0]/180*pi
  Constant5 : Constant  Value=[0 0 0]/180*pi
  Demux{1..6} (6 alike) : Demux  Outputs=3
  MATLAB Function1 : MATLAB Function  TreatAsAtomicUnit=on
  MATLAB Function2 : MATLAB Function  TreatAsAtomicUnit=on
  MATLAB Function3 : MATLAB Function  TreatAsAtomicUnit=on
  Product{1..4,6..7} (6 alike) : Product  Multiplication=Matrix(*)
  Rotation Angles to Direction Cosine Matrix : Angle2Dcm  rotationOrder=XYZ
      settings: AttributesFormatString=Rotation Order: %<rotationOrder>
  Rotation Angles to Direction Cosine Matrix1 : Angle2Dcm  rotationOrder=XYZ
      settings: AttributesFormatString=Rotation Order: %<rotationOrder>
  Rotation Angles to Direction Cosine Matrix2 : Angle2Dcm  rotationOrder=XYZ
      settings: AttributesFormatString=Rotation Order: %<rotationOrder>
  Selector1 : Selector  NumberOfDimensions=2  InputPortWidth=3  IndexOptions=Select all,Index vector (dialog)  Indices=[1:6],[surface_nodes.v_tail_joint.node_id]  OutputSizes=1,1
  Selector10 : Selector  NumberOfDimensions=2  InputPortWidth=3  IndexOptions=Index vector (dialog),Select all  Indices=[4:6],[surface_nodes.wing_R.node_id]  OutputSizes=1,1
  Selector11 : Selector  NumberOfDimensions=2  InputPortWidth=3  IndexOptions=Index vector (dialog),Select all  Indices=[4:6],[surface_nodes.wing_R.node_id]  OutputSizes=1,1
  Selector12 : Selector  NumberOfDimensions=2  InputPortWidth=3  IndexOptions=Index vector (dialog),Select all  Indices=[1:3],[surface_nodes.wing_R.node_id]  OutputSizes=1,1
  Selector13 : Selector  NumberOfDimensions=2  InputPortWidth=3  IndexOptions=Index vector (dialog),Select all  Indices=[4:6],[surface_nodes.wing_R.node_id]  OutputSizes=1,1
  Selector14 : Selector  NumberOfDimensions=2  InputPortWidth=3  IndexOptions=Index vector (dialog),Select all  Indices=[1:3],[surface_nodes.wing_R.node_id]  OutputSizes=1,1
  Selector2 : Selector  NumberOfDimensions=2  InputPortWidth=3  IndexOptions=Select all,Index vector (dialog)  Indices=[1:6],[surface_nodes.wing_joint.node_id]  OutputSizes=1,1
  Selector3 : Selector  NumberOfDimensions=2  InputPortWidth=3  IndexOptions=Select all,Index vector (dialog)  Indices=[1:6],[surface_nodes.wing_joint.node_id]  OutputSizes=1,1
  Selector4 : Selector  NumberOfDimensions=2  InputPortWidth=3  IndexOptions=Select all,Index vector (dialog)  Indices=[1:6],[surface_nodes.v_tail_joint.node_id]  OutputSizes=1,1
  Selector5 : Selector  NumberOfDimensions=2  InputPortWidth=3  IndexOptions=Select all,Index vector (dialog)  Indices=[1:6],surface_nodes.tail_bay.node_id  OutputSizes=1,1
  Selector6 : Selector  NumberOfDimensions=2  InputPortWidth=3  IndexOptions=Select all,Index vector (dialog)  Indices=[1:6],surface_nodes.tail_bay.node_id  OutputSizes=1,1
  Selector9 : Selector  NumberOfDimensions=2  InputPortWidth=3  IndexOptions=Index vector (dialog),Select all  Indices=[1:3],[surface_nodes.wing_R.node_id]  OutputSizes=1,1
  W_aero_station : Outport
  wires:
  Bus Creator3/1 -> W_aero_station/1
  Bus Creator2/1 -> Bus Creator3/3
  Bus Creator1/1 -> Bus Creator3/2
  Bus Creator/1 -> Bus Creator3/1
  Demux6/3 -> Bus Creator2/6  "Bending_momenty"
  Product3/1 -> Demux3/1
  Demux3/2 -> Bus Creator2/2  "shear_forcey"
  Demux3/3 -> Bus Creator2/3  "shear_forcez"
  Demux3/1 -> Bus Creator2/1  "Axial_Force"
  Demux6/2 -> Bus Creator2/5  "Bending_momentx"
  Demux6/1 -> Bus Creator2/4  "Torision_moment"
  Product4/1 -> Demux6/1
  Product2/1 -> Demux2/1
  Demux2/1 -> Bus Creator1/4  "Torision_moment"
  Demux2/2 -> Bus Creator1/5  "Bending_momentx"
  Demux1/1 -> Bus Creator1/1  "Axial_Force"
  Demux1/3 -> Bus Creator1/3  "shear_forcez"
  Demux1/2 -> Bus Creator1/2  "shear_forcey"
  Product1/1 -> Demux1/1
  Demux2/3 -> Bus Creator1/6  "Bending_momenty"
  Demux5/1 -> Bus Creator/4  "Torision_moment"
  Demux4/3 -> Bus Creator/3  "shear_forcez"
  Product6/1 -> Demux4/1
  Product7/1 -> Demux5/1
  Demux5/3 -> Bus Creator/6  "Bending_momenty"
  Demux4/2 -> Bus Creator/2  "shear_forcey"
  Demux5/2 -> Bus Creator/5  "Bending_momentx"
  Demux4/1 -> Bus Creator/1  "Axial_Force"
  Selector14/1 -> MATLAB Function3/1(F)
  Selector13/1 -> MATLAB Function3/2(M)
  Selector5/1 -> Selector14/1, Selector13/1
  Selector1/1 -> Selector12/1, Selector11/1
  Selector11/1 -> MATLAB Function2/2(M)
  Selector12/1 -> MATLAB Function2/1(F)
  Selector2/1 -> Selector9/1, Selector10/1
  Selector9/1 -> MATLAB Function1/1(F)
  Selector10/1 -> MATLAB Function1/2(M)
  Constant5/1 -> Rotation Angles to Direction Cosine Matrix/1
  MATLAB Function1/1(F_b) -> Product6/2
  Selector3/1 -> MATLAB Function1/3(r)
  Constant/1 -> MATLAB Function1/4(p)
  Rotation Angles to Direction Cosine Matrix/1 -> Product7/1, Product6/1
  MATLAB Function1/2(M_b) -> Product7/2
  MATLAB Function2/2(M_b) -> Product2/2
  Rotation Angles to Direction Cosine Matrix1/1 -> Product1/1, Product2/1
  Constant1/1 -> MATLAB Function2/4(p)
  Selector4/1 -> MATLAB Function2/3(r)
  MATLAB Function2/1(F_b) -> Product1/2
  Constant2/1 -> Rotation Angles to Direction Cosine Matrix1/1
  Constant4/1 -> Rotation Angles to Direction Cosine Matrix2/1
  MATLAB Function3/1(F_b) -> Product3/2
  Selector6/1 -> MATLAB Function3/3(r)
  Constant3/1 -> MATLAB Function3/4(p)
  Rotation Angles to Direction Cosine Matrix2/1 -> Product4/1, Product3/1
  MATLAB Function3/2(M_b) -> Product4/2
  Wb_total/1 -> Selector5/1, Selector1/1, Selector2/1
  r_cg_up/1 -> Selector3/1, Selector4/1, Selector6/1

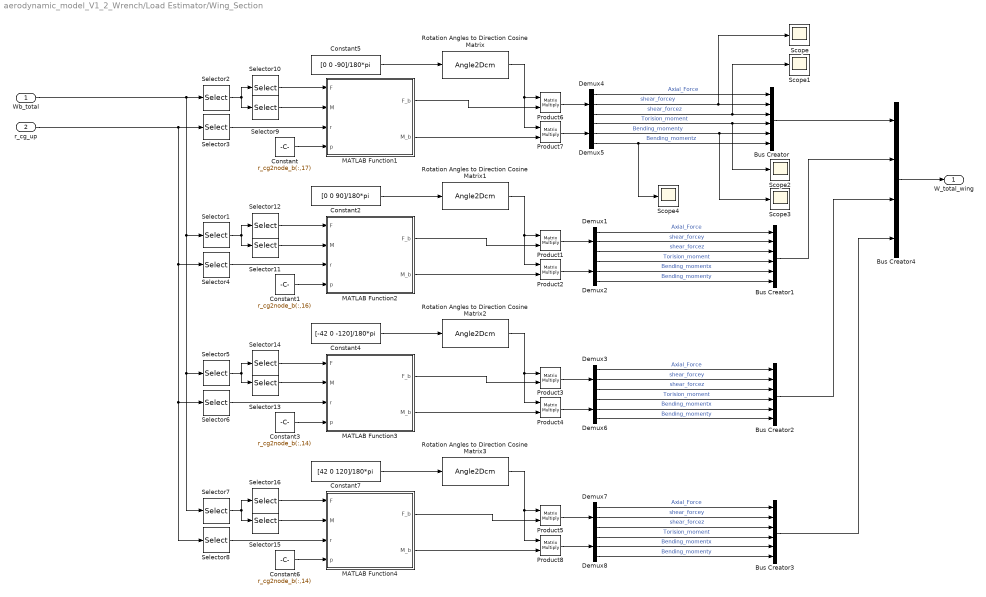
== system aerodynamic_model_V1_2_Wrench/Load Estimator/Wing_Section ==
  Wb_total : Inport
  r_cg_up : Inport  Port=2
  Bus Creator{,1..3} (4 alike) : BusCreator  Inputs=6
  Bus Creator4 : BusCreator  Inputs=4
  Constant : Constant  Value=r_cg2node_b(:,17)
  Constant1 : Constant  Value=r_cg2node_b(:,16)
  Constant2 : Constant  Value=[0 0 90]/180*pi
  Constant3 : Constant  Value=r_cg2node_b(:,14)
  Constant4 : Constant  Value=[-42 0 -120]/180*pi
  Constant5 : Constant  Value=[0 0 -90]/180*pi
  Constant6 : Constant  Value=r_cg2node_b(:,14)
  Constant7 : Constant  Value=[42 0 120]/180*pi
  Demux{1..8} (8 alike) : Demux  Outputs=3
  MATLAB Function1 : MATLAB Function  TreatAsAtomicUnit=on
  MATLAB Function2 : MATLAB Function  TreatAsAtomicUnit=on
  MATLAB Function3 : MATLAB Function  TreatAsAtomicUnit=on
  MATLAB Function4 : MATLAB Function  TreatAsAtomicUnit=on
  Product{1..8} (8 alike) : Product  Multiplication=Matrix(*)
  Rotation Angles to Direction Cosine Matrix{,1..3} (4 alike) : Angle2Dcm  rotationOrder=XYZ
      settings: AttributesFormatString=Rotation Order: %<rotationOrder>
  Scope{,1..4} (5 alike) : Scope
      Scope settings: ActiveDisplayYMinimum=-701.70070889117164  ActiveDisplayYMaximum=2692.587568384824  DataLoggingVariableName=ScopeData3
      Scope1 settings: ActiveDisplayYMinimum=-5860.8762190817188  ActiveDisplayYMaximum=-5388.1734134448989  DataLoggingVariableName=ScopeData4
      Scope2 settings: ActiveDisplayYMinimum=-1  ActiveDisplayYMaximum=1  DataLoggingVariableName=ScopeData5
      Scope3 settings: ActiveDisplayYMinimum=-45751.57172735683  ActiveDisplayYMaximum=65131.541259439364  DataLoggingVariableName=ScopeData6
      Scope4 settings: ActiveDisplayYMinimum=-1  ActiveDisplayYMaximum=1  DataLoggingVariableName=ScopeData7
  Selector1 : Selector  NumberOfDimensions=2  InputPortWidth=3  IndexOptions=Select all,Index vector (dialog)  Indices=[1:6],[surface_nodes.wing_R.node_id]  OutputSizes=1,1
  Selector{10,12,14,16} (4 alike) : Selector  NumberOfDimensions=2  InputPortWidth=3  IndexOptions=Index vector (dialog),Select all  Indices=[1:3],[surface_nodes.wing_R.node_id]  OutputSizes=1,1
  Selector{9,11,13,15} (4 alike) : Selector  NumberOfDimensions=2  InputPortWidth=3  IndexOptions=Index vector (dialog),Select all  Indices=[4:6],[surface_nodes.wing_R.node_id]  OutputSizes=1,1
  Selector2 : Selector  NumberOfDimensions=2  InputPortWidth=3  IndexOptions=Select all,Index vector (dialog)  Indices=[1:6],[surface_nodes.wing_L.node_id]  OutputSizes=1,1
  Selector3 : Selector  NumberOfDimensions=2  InputPortWidth=3  IndexOptions=Select all,Index vector (dialog)  Indices=[1:6],[surface_nodes.wing_L.node_id]  OutputSizes=1,1
  Selector4 : Selector  NumberOfDimensions=2  InputPortWidth=3  IndexOptions=Select all,Index vector (dialog)  Indices=[1:6],[surface_nodes.wing_R.node_id]  OutputSizes=1,1
  Selector5 : Selector  NumberOfDimensions=2  InputPortWidth=3  IndexOptions=Select all,Index vector (dialog)  Indices=[1:6],[surface_nodes.v_tail_L.node_id]  OutputSizes=1,1
  Selector6 : Selector  NumberOfDimensions=2  InputPortWidth=3  IndexOptions=Select all,Index vector (dialog)  Indices=[1:6],[surface_nodes.v_tail_L.node_id]  OutputSizes=1,1
  Selector7 : Selector  NumberOfDimensions=2  InputPortWidth=3  IndexOptions=Select all,Index vector (dialog)  Indices=[1:6],[surface_nodes.v_tail_R.node_id]  OutputSizes=1,1
  Selector8 : Selector  NumberOfDimensions=2  InputPortWidth=3  IndexOptions=Select all,Index vector (dialog)  Indices=[1:6],[surface_nodes.v_tail_R.node_id]  OutputSizes=1,1
  W_total_wing : Outport
  wires:
  Constant5/1 -> Rotation Angles to Direction Cosine Matrix/1
  MATLAB Function1/1(F_b) -> Product6/2
  Selector3/1 -> MATLAB Function1/3(r)
  Rotation Angles to Direction Cosine Matrix/1 -> Product7/1, Product6/1
  MATLAB Function1/2(M_b) -> Product7/2
  MATLAB Function2/2(M_b) -> Product2/2
  Rotation Angles to Direction Cosine Matrix1/1 -> Product1/1, Product2/1
  Constant1/1 -> MATLAB Function2/4(p)
  Selector4/1 -> MATLAB Function2/3(r)
  MATLAB Function2/1(F_b) -> Product1/2
  Constant2/1 -> Rotation Angles to Direction Cosine Matrix1/1
  Constant4/1 -> Rotation Angles to Direction Cosine Matrix2/1
  MATLAB Function3/1(F_b) -> Product3/2
  Selector6/1 -> MATLAB Function3/3(r)
  Constant3/1 -> MATLAB Function3/4(p)
  Rotation Angles to Direction Cosine Matrix2/1 -> Product4/1, Product3/1
  MATLAB Function3/2(M_b) -> Product4/2
  Wb_total/1 -> Selector1/1, Selector5/1, Selector7/1, Selector2/1
  r_cg_up/1 -> Selector8/1, Selector6/1, Selector4/1, Selector3/1
  MATLAB Function4/2(M_b) -> Product8/2
  Rotation Angles to Direction Cosine Matrix3/1 -> Product5/1, Product8/1
  Constant6/1 -> MATLAB Function4/4(p)
  Selector8/1 -> MATLAB Function4/3(r)
  MATLAB Function4/1(F_b) -> Product5/2
  Constant7/1 -> Rotation Angles to Direction Cosine Matrix3/1
  Product6/1 -> Demux4/1
  Product7/1 -> Demux5/1
  Product1/1 -> Demux1/1
  Product2/1 -> Demux2/1
  Selector12/1 -> MATLAB Function2/1(F)
  Selector11/1 -> MATLAB Function2/2(M)
  Selector1/1 -> Selector11/1, Selector12/1
  Selector5/1 -> Selector13/1, Selector14/1
  Selector13/1 -> MATLAB Function3/2(M)
  Selector14/1 -> MATLAB Function3/1(F)
  Selector7/1 -> Selector15/1, Selector16/1
  Selector15/1 -> MATLAB Function4/2(M)
  Selector16/1 -> MATLAB Function4/1(F)
  Demux4/2 -> Scope/1, Bus Creator/2  "shear_forcey"
  Demux4/3 -> Scope1/1, Bus Creator/3  "shear_forcez"
  Demux5/1 -> Scope2/1, Bus Creator/4  "Torision_moment"
  Demux5/2 -> Scope3/1, Bus Creator/5  "Bending_momenty"
  Demux5/3 -> Scope4/1, Bus Creator/6  "Bending_momentz"
  Demux4/1 -> Bus Creator/1  "Axial_Force"
  Demux1/1 -> Bus Creator1/1  "Axial_Force"
  Demux2/2 -> Bus Creator1/5  "Bending_momentx"
  Demux1/2 -> Bus Creator1/2  "shear_forcey"
  Demux2/3 -> Bus Creator1/6  "Bending_momenty"
  Demux1/3 -> Bus Creator1/3  "shear_forcez"
  Demux2/1 -> Bus Creator1/4  "Torision_moment"
  Demux6/1 -> Bus Creator2/4  "Torision_moment"
  Demux6/3 -> Bus Creator2/6  "Bending_momenty"
  Demux3/3 -> Bus Creator2/3  "shear_forcez"
  Demux3/1 -> Bus Creator2/1  "Axial_Force"
  Demux6/2 -> Bus Creator2/5  "Bending_momentx"
  Demux3/2 -> Bus Creator2/2  "shear_forcey"
  Product4/1 -> Demux6/1
  Product3/1 -> Demux3/1
  Product5/1 -> Demux7/1
  Demux7/3 -> Bus Creator3/3  "shear_forcez"
  Demux8/3 -> Bus Creator3/6  "Bending_momenty"
  Demux8/2 -> Bus Creator3/5  "Bending_momentx"
  Product8/1 -> Demux8/1
  Demux7/2 -> Bus Creator3/2  "shear_forcey"
  Demux8/1 -> Bus Creator3/4  "Torision_moment"
  Demux7/1 -> Bus Creator3/1  "Axial_Force"
  Bus Creator/1 -> Bus Creator4/1
  Bus Creator1/1 -> Bus Creator4/2
  Bus Creator2/1 -> Bus Creator4/3
  Bus Creator3/1 -> Bus Creator4/4
  Bus Creator4/1 -> W_total_wing/1
  Constant/1 -> MATLAB Function1/4(p)
  Selector2/1 -> Selector10/1, Selector9/1
  Selector10/1 -> MATLAB Function1/1(F)
  Selector9/1 -> MATLAB Function1/2(M)
